simulink model "y_mess_PI"  (R2026b)
settings: Solver=FixedStepAuto  StopTime=300  FixedStep=0.001
libraries: slpidlib x1
settings Model: SimulationMode=accelerator  Creator=Enrico  LastModifiedBy=Enrico

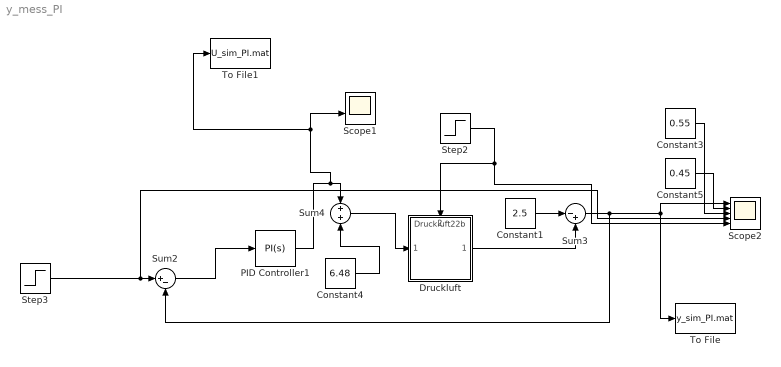
== system y_mess_PI ==
  Constant1 : Constant  Value=2.5
  Constant3 : Constant  Value=0.55
  Constant4 : Constant  Value=6.48
  Constant5 : Constant  Value=0.45
  Druckluft : ModelReference  InitFcn=set_param(gcs,'EnablePacing', 'on')  ModelNameDialog=Druckluft22b.slxp  ParameterArgumentNames=v  ParameterArgumentValues=v  UsingDefaultArgumentValue=0  ModelReferenceVersion=2.4  CopyOfModelProtected=on  v=3
      settings: PortSchema="{\"entries\":[{\"content\":{\"sides\":[{\"content\":{\"connectorIds\":[\"In1\"]},\"type\":\"ConnectorPlacement.EquallySpacedRectSide\",\"uuid\":\"9f5606e0-dfd9-4acc-b8ca-40de96c49444\"},{\"content\":{\"connectorIds\":[\"Out1\"],\"side\":\"RIGHT\"},\"type\":\"ConnectorPlacement.EquallySpacedRectSide\",\"uuid\":\"e73210b7-b638-4f03-9af5-56d1e88d4e70\"},{\"content\":{\"connectorIds\":[\"In2\"],\"side\":\"TOP\"},\"type\":\"ConnectorPlacement.EquallySpacedRectSide\",\"uuid\":\"b4caa743-0e25-4d8b-adf7-d97666dc0794\"}]},\"type\":\"ConnectorPlacement.EquallySpacedConnector\",\"uuid\":\"e51ec611-1b81-4c82-823b-92f4e9cc5570\"}],\"packageUris\":[\"http://schema.mathworks.com/mf0/Connector/R2020b\"],\"version\":\"1.0\"}"
  PID Controller1 : slpidlib/PID Controller  Controller=PI  Form=Parallel  TimeDomain=Continuous-time  UseExternalTs=off  SampleTime=-1  IntegratorMethod=Forward Euler  FilterMethod=Forward Euler  ControllerParametersSource=internal  P=4.85  I=0.67  UseKiTs=off  D=0  UseExternalDerivativeSource=off  N=100  UseFilter=on  TunerSelectOption=Transfer Function Based (PID Tuner App)  InitialConditionSource=internal  InitialConditionForIntegrator=0  InitialConditionForFilter=0  DifferentiatorICPrevScaledInput=0  ExternalReset=none  TrackingMode=off  Kt=1  LimitOutput=off  SatLimitsSource=internal  UpperSaturationLimit=inf  LowerSaturationLimit=-inf  LinearizeAsGain=on  AntiWindupMode=none  Kb=1  LimitIntegrator=off  UpperIntegratorSaturationLimit=inf  LowerIntegratorSaturationLimit=-inf  POutMin=[]  POutMax=[]  IOutMin=[]  IOutMax=[]  DOutMin=[]  DOutMax=[]  NOutMin=[]  NOutMax=[]  SumOutMin=[]  SumOutMax=[]  SaturationOutMin=[]  SaturationOutMax=[]  PParamMin=[]  PParamMax=[]  IParamMin=[]  IParamMax=[]  DParamMin=[]  DParamMax=[]  NParamMin=[]  NParamMax=[]  KbParamMin=[]  KbParamMax=[]  KtParamMin=[]  KtParamMax=[]  KbOutMin=[]  KbOutMax=[]  KtOutMin=[]  KtOutMax=[]  IntegratorOutMin=[]  IntegratorOutMax=[]  FilterOutMin=[]  FilterOutMax=[]  SumI1OutMin=[]  SumI1OutMax=[]  SumI2OutMin=[]  SumI2OutMax=[]  SumI3OutMin=[]  SumI3OutMax=[]  SumI4OutMin=[]  SumI4OutMax=[]  SumDOutMin=[]  SumDOutMax=[]  DifferentiatorOutMin=[]  DifferentiatorOutMax=[]  FilterDiffOutCoefMin=[]  FilterDiffOutCoefMax=[]  ReciprocalOutMin=[]  ReciprocalOutMax=[]  SumDenOutMin=[]  SumDenOutMax=[]  SumNumOutMin=[]  SumNumOutMax=[]  DivideOutMin=[]  DivideOutMax=[]  UdiffTsProdOutMin=[]  UdiffTsProdOutMax=[]  NTsProdOutMin=[]  NTsProdOutMax=[]  UintegralTsProdOutMin=[]  UintegralTsProdOutMax=[]  UngainTsProdOutMin=[]  UngainTsProdOutMax=[]  ClampingZeroOutDataTypeStr=Inherit: Inherit via back propagation  ClampingZeroOutMin=[]  ClampingZeroOutMax=[]  FilterDenConstantOutDataTypeStr=Inherit: Inherit via back propagation  FilterDenConstantOutMin=[]  FilterDenConstantOutMax=[]  PCopyOutDataTypeStr=Inherit: Inherit via back propagation  PCopyOutMin=[]  PCopyOutMax=[]  NCopyOutDataTypeStr=Inherit: Inherit via back propagation  NCopyOutMin=[]  NCopyOutMax=[]  IntegratorContinuousStateAttributes=''  IntegratorStateMustResolveToSignalObject=off  IntegratorRTWStateStorageClass=Auto  FilterContinuousStateAttributes=''  FilterStateMustResolveToSignalObject=off  FilterRTWStateStorageClass=Auto  ParallelPVariant=InternalParameters  IdealPVariant=Disabled  IVariant=InternalParameters  DVariant=Disabled  IntegratorVariant=Continuous  SatVariant=Disabled  AWVariant=Passthrough  PCopyVariant=Disabled  TRVariant=Disabled  FdbkBlocksVariant=Forward  IdealPFdbkVariant=Disabled  SatFdbkVariant=Disabled  DerivativeFilterVariant=Disabled  NVariant=Disabled  NCopyVariant=Disabled_SignalSpec  FilterICVariant=Disabled  IntegratorICVariant=InternalICs  ExternalResetVariant=Disabled  TRSumVariant=Passthrough  SumFdbkVariant=Disabled  SumVariant=Sum_PI  TsampFilterVariant=InternalTs  TsampNgainVariant=Passthrough  TsampIntegralVariant=Disabled_SignalSpec  ExternalSaturationOutDataTypeStr=Inherit: Same as second input  DerivativeSourceVariant=Disabled  PreIntVariant=InternalPreInt
  Scope1 : Scope  NumInputPorts=5
      settings: ActiveDisplayYMinimum=-6.6880065887485625  ActiveDisplayYMaximum=7.943111843194286  DataLoggingMaxPoints=100000
  Scope2 : Scope  NumInputPorts=5
      settings: ActiveDisplayYMinimum=0.17266164412219304  ActiveDisplayYMaximum=0.68182277236579525  DataLoggingMaxPoints=100000  DataLoggingVariableName=ScopeData2
  Step2 : Step  Time=200  FinalValue=0.5  SampleTime=0
  Step3 : Step  Time=100  FinalValue=0.5  SampleTime=0
  Sum2 : Sum  Inputs=|+-
  Sum3 : Sum  Inputs=|-+
  Sum4 : Sum
  To File : ToFile  Filename=y_sim_PI.mat  MatrixName=y_sim_PI  SaveFormat=Timeseries
  To File1 : ToFile  Filename=U_sim_PI.mat  MatrixName=y_sim_PI  SaveFormat=Timeseries
  wires:
  Constant4/1 -> Sum4/2
  Druckluft/1 -> Sum3/2
  Sum3/1 -> Scope2/1, To File/1, Sum2/2
  Step2/1 -> Scope2/5, Druckluft/2
  PID Controller1/1 -> To File1/1, Scope1/4, Sum4/1
  Constant3/1 -> Scope2/3
  Step3/1 -> Scope2/4, Sum2/1
  Sum2/1 -> PID Controller1/1
  Constant5/1 -> Scope2/2
  Sum4/1 -> Druckluft/1
  Constant1/1 -> Sum3/1
